simulink model "model_file_sim"  (R2025b)
settings: Solver=ode4  StartTime=0.0  StopTime=5000  FixedStep=1  RelTol=1e-3
values from neighbouring files (symbols this model uses):
  Rc_alu = 10    [modele_valeur.m]
  Rc_fan = 1.2/2    (= 0.6)    [modele_valeur.m]
  Rc_fan1 = 1.2/2    (= 0.6)    [modele_valeur.m]
  Rc_pet = 20/2    (= 10)    [modele_valeur.m]
  Rc_pet1 = 20/2    (= 10)    [modele_valeur.m]
  Rth_alu = 0.1/2    (= 0.05)    [modele_valeur.m]
  Rth_alu2 = 0.1/2    (= 0.05)    [modele_valeur.m]
  Rth_fan = 2.5/2    (= 1.25)    [modele_valeur.m]
  Rth_fan2 = 2.5/2    (= 1.25)    [modele_valeur.m]
  Rth_pet = 5/2    (= 2.5)    [modele_valeur.m]
  Rth_pet2 = 5/2    (= 2.5)    [modele_valeur.m]
  Rth_sen = 24    [modele_valeur.m]
  Rv = 50    [modele_valeur.m]
  Ts = 1    [model_file_elec.m]    (also in modele_valeur.m; thermal_rl_env.m = 0.5)
libraries: fl_lib x34, nesl_utility x6, slpidlib x1, eeAlternativeControllers x1, simulink x1
settings Model: Creator=33683  LastModifiedBy=nael
settings DataIOCC: ExternalInput=data_in  LoadExternalInput=on  SaveOutput=off  SignalLogging=off  DSMLogging=off  SaveTime=off  ReturnWorkspaceOutputs=off
settings SimscapeCC: ExplicitSolverDiagnosticOptions=none

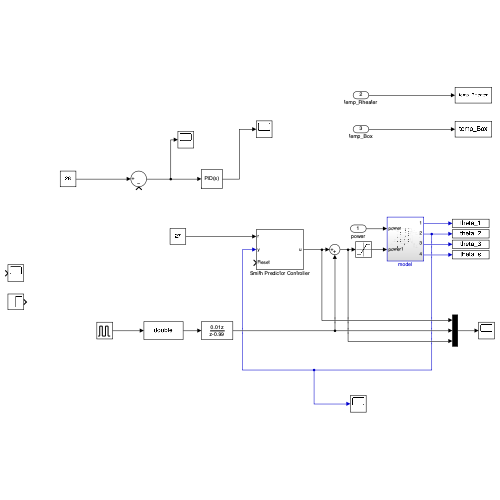
[thumbnail: Simulink's stored preview of the top-level diagram]
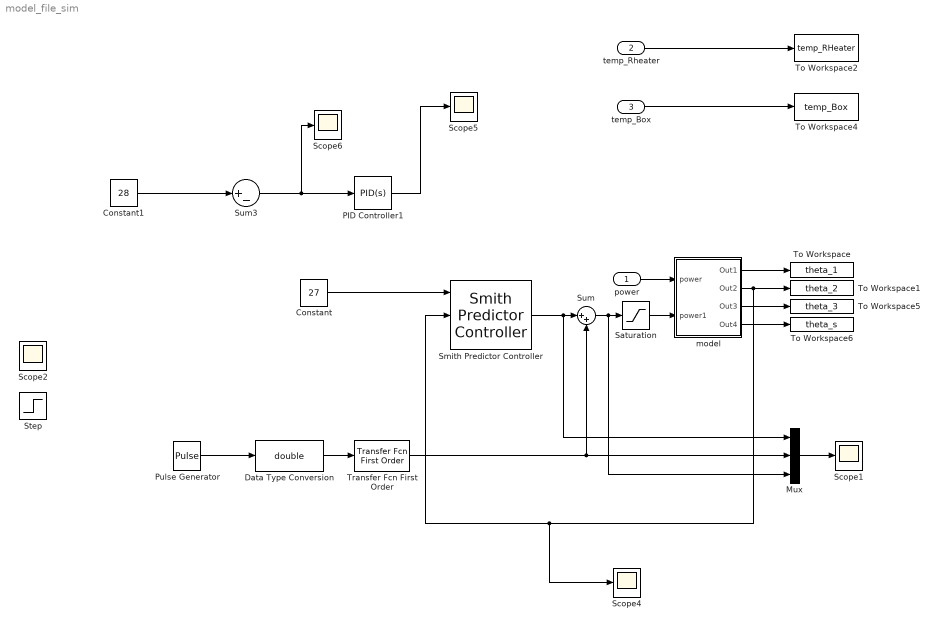
== system model_file_sim ==
  power : Inport
  temp_Rheater : Inport  Port=2
  temp_Box : Inport  Port=3
  Constant : Constant  Value=27
  Constant1 : Constant  Value=28
  Data Type Conversion : DataTypeConversion  OutDataTypeStr=double  SaturateOnIntegerOverflow=off  RndMeth=Floor
  Mux : Mux  Inputs=3
  PID Controller1 : slpidlib/PID Controller  Controller=PID  Form=Parallel  TimeDomain=Continuous-time  UseExternalTs=off  SampleTime=Ts  IntegratorMethod=Forward Euler  FilterMethod=Forward Euler  ControllerParametersSource=internal  P=3  I=0.05  UseKiTs=off  D=0  UseExternalDerivativeSource=off  N=10  UseFilter=on  TunerSelectOption=Transfer Function Based (PID Tuner App)  InitialConditionSource=internal  InitialConditionForIntegrator=0  InitialConditionForFilter=0  DifferentiatorICPrevScaledInput=0  ExternalReset=none  TrackingMode=off  Kt=1  LimitOutput=off  SatLimitsSource=internal  UpperSaturationLimit=inf  LowerSaturationLimit=-inf  LinearizeAsGain=on  AntiWindupMode=none  Kb=1  LimitIntegrator=off  UpperIntegratorSaturationLimit=inf  LowerIntegratorSaturationLimit=-inf  POutMin=[]  POutMax=[]  IOutMin=[]  IOutMax=[]  DOutMin=[]  DOutMax=[]  NOutMin=[]  NOutMax=[]  SumOutMin=[]  SumOutMax=[]  SaturationOutMin=[]  SaturationOutMax=[]  PParamMin=[]  PParamMax=[]  IParamMin=[]  IParamMax=[]  DParamMin=[]  DParamMax=[]  NParamMin=[]  NParamMax=[]  KbParamMin=[]  KbParamMax=[]  KtParamMin=[]  KtParamMax=[]  KbOutMin=[]  KbOutMax=[]  KtOutMin=[]  KtOutMax=[]  IntegratorOutMin=[]  IntegratorOutMax=[]  FilterOutMin=[]  FilterOutMax=[]  SumI1OutMin=[]  SumI1OutMax=[]  SumI2OutMin=[]  SumI2OutMax=[]  SumI3OutMin=[]  SumI3OutMax=[]  SumI4OutMin=[]  SumI4OutMax=[]  SumDOutMin=[]  SumDOutMax=[]  DifferentiatorOutMin=[]  DifferentiatorOutMax=[]  FilterDiffOutCoefMin=[]  FilterDiffOutCoefMax=[]  ReciprocalOutMin=[]  ReciprocalOutMax=[]  SumDenOutMin=[]  SumDenOutMax=[]  SumNumOutMin=[]  SumNumOutMax=[]  DivideOutMin=[]  DivideOutMax=[]  UdiffTsProdOutMin=[]  UdiffTsProdOutMax=[]  NTsProdOutMin=[]  NTsProdOutMax=[]  UintegralTsProdOutMin=[]  UintegralTsProdOutMax=[]  UngainTsProdOutMin=[]  UngainTsProdOutMax=[]  ClampingZeroOutDataTypeStr=Inherit: Inherit via back propagation  ClampingZeroOutMin=[]  ClampingZeroOutMax=[]  FilterDenConstantOutDataTypeStr=Inherit: Inherit via back propagation  FilterDenConstantOutMin=[]  FilterDenConstantOutMax=[]  PCopyOutDataTypeStr=Inherit: Inherit via back propagation  PCopyOutMin=[]  PCopyOutMax=[]  NCopyOutDataTypeStr=Inherit: Inherit via back propagation  NCopyOutMin=[]  NCopyOutMax=[]  IntegratorContinuousStateAttributes=''  IntegratorStateMustResolveToSignalObject=off  IntegratorRTWStateStorageClass=Auto  FilterContinuousStateAttributes=''  FilterStateMustResolveToSignalObject=off  FilterRTWStateStorageClass=Auto  ParallelPVariant=InternalParameters  IdealPVariant=Disabled  IVariant=InternalParameters  DVariant=InternalParameters  IntegratorVariant=Continuous  SatVariant=Disabled  AWVariant=Passthrough  PCopyVariant=Disabled  TRVariant=Disabled  FdbkBlocksVariant=Forward  IdealPFdbkVariant=Disabled  SatFdbkVariant=Disabled  DerivativeFilterVariant=ContFilter  NVariant=InternalParameters  NCopyVariant=Disabled  FilterICVariant=InternalICsFilter  IntegratorICVariant=InternalICs  ExternalResetVariant=Disabled  TRSumVariant=Passthrough  SumFdbkVariant=Disabled  SumVariant=Sum_PID  TsampFilterVariant=InternalTs  TsampNgainVariant=Passthrough  TsampIntegralVariant=Disabled_SignalSpec  ExternalSaturationOutDataTypeStr=Inherit: Same as second input  DerivativeSourceVariant=ErrorSignal  PreIntVariant=InternalPreInt
  Pulse Generator : DiscretePulseGenerator  PulseType=Time based  Amplitude=2  Period=100  PulseWidth=20  PhaseDelay=100
  Saturation : Saturate  UpperLimit=50  LowerLimit=0
  Scope{1..2,4..6} (5 alike) : Scope
      Scope1 settings: ActiveDisplayYMinimum=-0.696783783226232  ActiveDisplayYMaximum=6.2710540490360893  DataLoggingVariableName=ScopeData2
      Scope2 settings: ActiveDisplayYMinimum=-3.19147364275E+6  ActiveDisplayYMaximum=2.865654132791E+7
      Scope4 settings: ActiveDisplayYMinimum=21.349467164172967  ActiveDisplayYMaximum=27.854795522443293
      Scope5 settings: ActiveDisplayYMinimum=-12.29216  ActiveDisplayYMaximum=133.10616  DataLoggingVariableName=ScopeData3
      Scope6 settings: ActiveDisplayYMinimum=-3.6781  ActiveDisplayYMaximum=7.07534  DataLoggingVariableName=ScopeData5
  Smith Predictor Controller : eeAlternativeControllers/Smith Predictor Controller  Kp=3  Ki=0.05  x0=0  B=5  A=0  numd=b  dend=a  d=1  Ts=Ts
      settings: LibrarySourceBlock=ee_sl_lib/General Control/Smith Predictor Controller
  Step : Step  Time=100  After=5  SampleTime=0
  Sum : Sum  Inputs=|++
  Sum3 : Sum  Inputs=|+-
  To Workspace : ToWorkspace  VariableName=theta_1  SampleTime=Ts
  To Workspace1 : ToWorkspace  VariableName=theta_2  SampleTime=Ts
  To Workspace2 : ToWorkspace  VariableName=temp_RHeater  SampleTime=Ts
  To Workspace4 : ToWorkspace  VariableName=temp_Box  SampleTime=Ts
  To Workspace5 : ToWorkspace  VariableName=theta_3  SampleTime=Ts
  To Workspace6 : ToWorkspace  VariableName=theta_s  SampleTime=Ts
  Transfer Fcn First Order : simulink/Discrete/Transfer Fcn First Order  PoleZ=0.99  ICPrevOutput=0.0  DoSatur=off
  model : Subsystem
  wires:
  temp_Rheater/1 -> To Workspace2/1
  temp_Box/1 -> To Workspace4/1
  model/1(Out1) -> To Workspace/1
  model/2(Out2) -> Scope4/1, Smith Predictor Controller/2, To Workspace1/1
  model/3(Out3) -> To Workspace5/1
  model/4(Out4) -> To Workspace6/1
  Sum3/1 -> Scope6/1, PID Controller1/1
  Constant/1 -> Smith Predictor Controller/1
  Constant1/1 -> Sum3/1
  PID Controller1/1 -> Scope5/1
  power/1 -> model/1(power)
  Sum/1 -> Mux/3, Saturation/1
  Mux/1 -> Scope1/1
  Transfer Fcn First Order/1 -> Sum/2, Mux/2
  Pulse Generator/1 -> Data Type Conversion/1
  Data Type Conversion/1 -> Transfer Fcn First Order/1
  Smith Predictor Controller/1 -> Mux/1, Sum/1
  Saturation/1 -> model/2(power1)

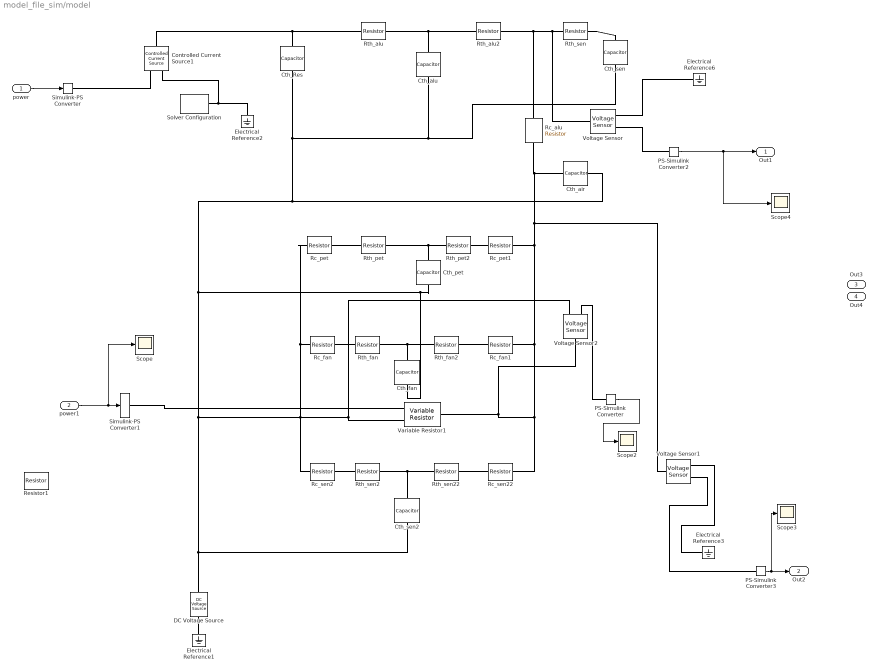
== system model_file_sim/model ==
  power : Inport
  power1 : Inport  Port=2
  Controlled Current Source1 : fl_lib/Electrical/Electrical Sources/Controlled Current Source
  Cth_Res : fl_lib/Electrical/Electrical Elements/Capacitor  c=Cth_Res F  r=0 Ohm  g=0 1/Ohm  i_specify=off  i_priority=None  i=0 A  i_nominal_specify=off  i_nominal_value=1  i_nominal_unit=A  v_specify=off  v_priority=None  v=0 V  v_nominal_specify=off  v_nominal_value=1  v_nominal_unit=V  vc_specify=off  vc_priority=High  vc=0 V  vc_nominal_specify=off  vc_nominal_value=1  vc_nominal_unit=V
  Cth_air : fl_lib/Electrical/Electrical Elements/Capacitor  c=Cth_air F  r=0 Ohm  g=0 1/Ohm  i_specify=off  i_priority=None  i=0 A  i_nominal_specify=off  i_nominal_value=1  i_nominal_unit=A  v_specify=off  v_priority=None  v=0 V  v_nominal_specify=off  v_nominal_value=1  v_nominal_unit=V  vc_specify=off  vc_priority=High  vc=0 V  vc_nominal_specify=off  vc_nominal_value=1  vc_nominal_unit=V
  Cth_alu : fl_lib/Electrical/Electrical Elements/Capacitor  c=Cth_alu F  r=0 Ohm  g=0 1/Ohm  i_specify=off  i_priority=None  i=0 A  i_nominal_specify=off  i_nominal_value=1  i_nominal_unit=A  v_specify=off  v_priority=None  v=0 V  v_nominal_specify=off  v_nominal_value=1  v_nominal_unit=V  vc_specify=off  vc_priority=High  vc=0 V  vc_nominal_specify=off  vc_nominal_value=1  vc_nominal_unit=V
  Cth_fan : fl_lib/Electrical/Electrical Elements/Capacitor  c=Cth_fan F  r=0 Ohm  g=0 1/Ohm  i_specify=off  i_priority=None  i=0 A  i_nominal_specify=off  i_nominal_value=1  i_nominal_unit=A  v_specify=off  v_priority=None  v=0 V  v_nominal_specify=off  v_nominal_value=1  v_nominal_unit=V  vc_specify=off  vc_priority=High  vc=0 V  vc_nominal_specify=off  vc_nominal_value=1  vc_nominal_unit=V
  Cth_pet : fl_lib/Electrical/Electrical Elements/Capacitor  c=Cth_pet F  r=0 Ohm  g=0 1/Ohm  i_specify=off  i_priority=None  i=0 A  i_nominal_specify=off  i_nominal_value=1  i_nominal_unit=A  v_specify=off  v_priority=None  v=0 V  v_nominal_specify=off  v_nominal_value=1  v_nominal_unit=V  vc_specify=off  vc_priority=High  vc=0 V  vc_nominal_specify=off  vc_nominal_value=1  vc_nominal_unit=V
  Cth_sen : fl_lib/Electrical/Electrical Elements/Capacitor  c=Cth_sen F  r=0 Ohm  g=0 1/Ohm  i_specify=off  i_priority=None  i=0 A  i_nominal_specify=off  i_nominal_value=1  i_nominal_unit=A  v_specify=off  v_priority=None  v=0 V  v_nominal_specify=off  v_nominal_value=1  v_nominal_unit=V  vc_specify=off  vc_priority=High  vc=0 V  vc_nominal_specify=off  vc_nominal_value=1  vc_nominal_unit=V
  Cth_sen2 : fl_lib/Electrical/Electrical Elements/Capacitor  c=Cth_pet F  r=0 Ohm  g=0 1/Ohm  i_specify=off  i_priority=None  i=0 A  i_nominal_specify=off  i_nominal_value=1  i_nominal_unit=A  v_specify=off  v_priority=None  v=0 V  v_nominal_specify=off  v_nominal_value=1  v_nominal_unit=V  vc_specify=off  vc_priority=High  vc=0 V  vc_nominal_specify=off  vc_nominal_value=1  vc_nominal_unit=V
  DC Voltage Source : fl_lib/Electrical/Electrical Sources/DC Voltage Source  v0=22 V
  Electrical Reference{1..3,6} (4 alike) : fl_lib/Electrical/Electrical Elements/Electrical Reference
  PS-Simulink Converter : nesl_utility/PS-Simulink Converter  PhysicalDomain=network_engine_domain  SubClassName=ps_output  LeftPortType=input  RightPortType=output  PseudoPeriodic=off  Frequencies=[]  VectorFormat=inherit  Unit=inherit  AffineConversion=off
  PS-Simulink Converter2 : nesl_utility/PS-Simulink Converter  PhysicalDomain=network_engine_domain  SubClassName=ps_output  LeftPortType=input  RightPortType=output  PseudoPeriodic=off  Frequencies=[]  VectorFormat=inherit  Unit=inherit  AffineConversion=off
  PS-Simulink Converter3 : nesl_utility/PS-Simulink Converter  PhysicalDomain=network_engine_domain  SubClassName=ps_output  LeftPortType=input  RightPortType=output  PseudoPeriodic=off  Frequencies=[]  VectorFormat=inherit  Unit=inherit  AffineConversion=off
  Rc_alu : fl_lib/Electrical/Electrical Elements/Resistor  R=Rc_alu Ohm  i_specify=off  i_priority=None  i=0 A  i_nominal_specify=off  i_nominal_value=1  i_nominal_unit=A  v_specify=off  v_priority=None  v=0 V  v_nominal_specify=off  v_nominal_value=1  v_nominal_unit=V
  Rc_fan : fl_lib/Electrical/Electrical Elements/Resistor  R=Rc_fan Ohm  i_specify=off  i_priority=None  i=0 A  i_nominal_specify=off  i_nominal_value=1  i_nominal_unit=A  v_specify=off  v_priority=None  v=0 V  v_nominal_specify=off  v_nominal_value=1  v_nominal_unit=V
  Rc_fan1 : fl_lib/Electrical/Electrical Elements/Resistor  R=Rc_fan1 Ohm  i_specify=off  i_priority=None  i=0 A  i_nominal_specify=off  i_nominal_value=1  i_nominal_unit=A  v_specify=off  v_priority=None  v=0 V  v_nominal_specify=off  v_nominal_value=1  v_nominal_unit=V
  Rc_pet : fl_lib/Electrical/Electrical Elements/Resistor  R=Rc_pet Ohm  i_specify=off  i_priority=None  i=0 A  i_nominal_specify=off  i_nominal_value=1  i_nominal_unit=A  v_specify=off  v_priority=None  v=0 V  v_nominal_specify=off  v_nominal_value=1  v_nominal_unit=V
  Rc_pet1 : fl_lib/Electrical/Electrical Elements/Resistor  R=Rc_pet1 Ohm  i_specify=off  i_priority=None  i=0 A  i_nominal_specify=off  i_nominal_value=1  i_nominal_unit=A  v_specify=off  v_priority=None  v=0 V  v_nominal_specify=off  v_nominal_value=1  v_nominal_unit=V
  Rc_sen2 : fl_lib/Electrical/Electrical Elements/Resistor  R=Rc_fan Ohm  i_specify=off  i_priority=None  i=0 A  i_nominal_specify=off  i_nominal_value=1  i_nominal_unit=A  v_specify=off  v_priority=None  v=0 V  v_nominal_specify=off  v_nominal_value=1  v_nominal_unit=V
  Rc_sen22 : fl_lib/Electrical/Electrical Elements/Resistor  R=Rth_fan Ohm  i_specify=off  i_priority=None  i=0 A  i_nominal_specify=off  i_nominal_value=1  i_nominal_unit=A  v_specify=off  v_priority=None  v=0 V  v_nominal_specify=off  v_nominal_value=1  v_nominal_unit=V
  Resistor1 : fl_lib/Electrical/Electrical Elements/Resistor  R=Rv Ohm  i_specify=off  i_priority=None  i=0 A  i_nominal_specify=off  i_nominal_value=1  i_nominal_unit=A  v_specify=off  v_priority=None  v=0 V  v_nominal_specify=off  v_nominal_value=1  v_nominal_unit=V
  Rth_alu : fl_lib/Electrical/Electrical Elements/Resistor  R=Rth_alu Ohm  i_specify=off  i_priority=None  i=0 A  i_nominal_specify=off  i_nominal_value=1  i_nominal_unit=A  v_specify=off  v_priority=None  v=0 V  v_nominal_specify=off  v_nominal_value=1  v_nominal_unit=V
  Rth_alu2 : fl_lib/Electrical/Electrical Elements/Resistor  R=Rth_alu2 Ohm  i_specify=off  i_priority=None  i=0 A  i_nominal_specify=off  i_nominal_value=1  i_nominal_unit=A  v_specify=off  v_priority=None  v=0 V  v_nominal_specify=off  v_nominal_value=1  v_nominal_unit=V
  Rth_fan : fl_lib/Electrical/Electrical Elements/Resistor  R=Rth_fan Ohm  i_specify=off  i_priority=None  i=0 A  i_nominal_specify=off  i_nominal_value=1  i_nominal_unit=A  v_specify=off  v_priority=None  v=0 V  v_nominal_specify=off  v_nominal_value=1  v_nominal_unit=V
  Rth_fan2 : fl_lib/Electrical/Electrical Elements/Resistor  R=Rth_fan2 Ohm  i_specify=off  i_priority=None  i=0 A  i_nominal_specify=off  i_nominal_value=1  i_nominal_unit=A  v_specify=off  v_priority=None  v=0 V  v_nominal_specify=off  v_nominal_value=1  v_nominal_unit=V
  Rth_pet : fl_lib/Electrical/Electrical Elements/Resistor  R=Rth_pet Ohm  i_specify=off  i_priority=None  i=0 A  i_nominal_specify=off  i_nominal_value=1  i_nominal_unit=A  v_specify=off  v_priority=None  v=0 V  v_nominal_specify=off  v_nominal_value=1  v_nominal_unit=V
  Rth_pet2 : fl_lib/Electrical/Electrical Elements/Resistor  R=Rth_pet2 Ohm  i_specify=off  i_priority=None  i=0 A  i_nominal_specify=off  i_nominal_value=1  i_nominal_unit=A  v_specify=off  v_priority=None  v=0 V  v_nominal_specify=off  v_nominal_value=1  v_nominal_unit=V
  Rth_sen : fl_lib/Electrical/Electrical Elements/Resistor  R=Rth_sen Ohm  i_specify=off  i_priority=None  i=0 A  i_nominal_specify=off  i_nominal_value=1  i_nominal_unit=A  v_specify=off  v_priority=None  v=0 V  v_nominal_specify=off  v_nominal_value=1  v_nominal_unit=V
  Rth_sen2 : fl_lib/Electrical/Electrical Elements/Resistor  R=Rth_fan Ohm  i_specify=off  i_priority=None  i=0 A  i_nominal_specify=off  i_nominal_value=1  i_nominal_unit=A  v_specify=off  v_priority=None  v=0 V  v_nominal_specify=off  v_nominal_value=1  v_nominal_unit=V
  Rth_sen22 : fl_lib/Electrical/Electrical Elements/Resistor  R=Rc_fan Ohm  i_specify=off  i_priority=None  i=0 A  i_nominal_specify=off  i_nominal_value=1  i_nominal_unit=A  v_specify=off  v_priority=None  v=0 V  v_nominal_specify=off  v_nominal_value=1  v_nominal_unit=V
  Scope{,2..4} (4 alike) : Scope
      Scope settings: ActiveDisplayYMinimum=1.1179174747738359  ActiveDisplayYMaximum=6.0694205759249709
      Scope2 settings: ActiveDisplayYMinimum=-0.6454786667977801  ActiveDisplayYMaximum=5.809308001180022
      Scope3 settings: ActiveDisplayYMinimum=21.048786988457906  ActiveDisplayYMaximum=30.56091710387885  DataLoggingVariableName=ScopeData2
      Scope4 settings: ActiveDisplayYMinimum=14.19123  ActiveDisplayYMaximum=92.27893  DataLoggingVariableName=ScopeData4
  Simulink-PS Converter : nesl_utility/Simulink-PS Converter  PhysicalDomain=network_engine_domain  SubClassName=ps_input  LeftPortType=input  RightPortType=output  PseudoPeriodic=off  Frequencies=[]  NoiseDistribution=none  NoiseParameters=[]  Unit=1  AffineConversion=off  FilteringAndDerivatives=provide  SimscapeFilterOrder=1  InputFilterTimeConstant=0.001  UdotUserProvided=0
  Simulink-PS Converter1 : nesl_utility/Simulink-PS Converter  PhysicalDomain=network_engine_domain  SubClassName=ps_input  LeftPortType=input  RightPortType=output  PseudoPeriodic=off  Frequencies=[]  NoiseDistribution=none  NoiseParameters=[]  Unit=V/A  AffineConversion=off  FilteringAndDerivatives=filter  SimscapeFilterOrder=1  InputFilterTimeConstant=Ts  UdotUserProvided=0
  Solver Configuration : nesl_utility/Solver Configuration  PhysicalDomain=network_engine_domain  SubClassName=solver  LeftPortType=input  RightPortType=generic  Tones=[]  Harmonics=[]  SimulateNoise=off  Profile=off  UseLocalSampling=off  EnableSwitchedLinearOptims=on  FrequencyDomain=off  UseCCode=off  RelTol=0.001  AbsTol=0.001  MinStep=1e-09  ToWorkspace=off  RevertToSquareIcSolve=off  NumHomotopyIterations=100  PhasorMode=off  PhasorModeNumHarmonics=1  ConsistencySolver=NEWTON_XTOL_AFTER_FTOL  IndexReductionMethod=DerivativeReplacement  DoDC=off  ResidualTolerance=1e-09  ConsistencyTolSource=GLOBAL  ConsistencyAbsTol=0.001  ConsistencyRelTol=0.001  ConsistencyTolFactor=0.001  UseLocalSolver=off  LocalSolverChoice=NE_BACKWARD_EULER_ADVANCER  ResolveIndetEquations=on  FunctionEvalNumThread=1  LocalSolverSampleTime=0.001  DoFixedCost=off  MaxNonlinIter=3  MaxModeIter=2  ComputeImpulses=off  ImpulseIterations=2  LinearAlgebra=auto  LinearAlgebraNumThread=0  EquationFormulation=NE_TIME_EF  DelaysMemoryBudget=1024  AutomaticFiltering=on  FilteringTimeConstant=0.001  PartitionStorageMethod=AS_NEEDED  PartitionMemoryBudget=1024  PartitionMethod=ROBUST  MultibodyUseLocalSolver=off  MultibodyLocalSolverChoice=ODE1  MultibodyLocalSolverSampleTime=0.001
  Variable Resistor1 : fl_lib/Electrical/Electrical Elements/Variable Resistor  Rmin=0.2 Ohm  thermalEnable=false  thermal_mass=1 J/K  i_specify=off  i_priority=None  i=0 A  i_nominal_specify=off  i_nominal_value=1  i_nominal_unit=A  v_specify=off  v_priority=None  v=0 V  v_nominal_specify=off  v_nominal_value=1  v_nominal_unit=V  T_specify=off  T_priority=None  T=300 K  T_nominal_specify=off  T_nominal_value=1  T_nominal_unit=K
  Voltage Sensor : fl_lib/Electrical/Electrical Sensors/Voltage Sensor
  Voltage Sensor1 : fl_lib/Electrical/Electrical Sensors/Voltage Sensor
  Voltage Sensor2 : fl_lib/Electrical/Electrical Sensors/Voltage Sensor
  Out1 : Outport
  Out2 : Outport  Port=2
  Out3 : Outport  Port=3
  Out4 : Outport  Port=4
  wires:
  PS-Simulink Converter3/1 -> Scope3/1, Out2/1
  PS-Simulink Converter2/1 -> Scope4/1, Out1/1
  power/1 -> Simulink-PS Converter/1
  PS-Simulink Converter/1 -> Scope2/1
  power1/1 -> Scope/1, Simulink-PS Converter1/1
  connections:
  Cth_Res/RConn1 -- Cth_sen/RConn1 -- Cth_alu/RConn1 -- Cth_air/RConn1 -- Cth_fan/RConn1 -- Cth_pet/RConn1 -- DC Voltage Source/LConn1 -- Cth_sen2/RConn1 -- Variable Resistor1/LConn2 -- Voltage Sensor2/RConn2 -- Rc_sen2/LConn1 -- Rc_pet/LConn1 -- Rc_fan/LConn1
  Voltage Sensor/LConn1 -- Rth_alu2/RConn1 -- Rc_alu/LConn1 -- Rth_sen/LConn1
  Rth_pet/RConn1 -- Cth_pet/LConn1 -- Rth_pet2/LConn1
  Rth_fan2/LConn1 -- Cth_fan/LConn1 -- Rth_fan/RConn1
  Cth_alu/LConn1 -- Rth_alu2/LConn1 -- Rth_alu/RConn1
  Cth_Res/LConn1 -- Controlled Current Source1/LConn1 -- Rth_alu/LConn1
  Solver Configuration/RConn1 -- Controlled Current Source1/RConn2 -- Electrical Reference2/LConn1
  Rth_sen22/LConn1 -- Rth_sen2/RConn1 -- Cth_sen2/LConn1
  Electrical Reference3/LConn1 -- Voltage Sensor1/RConn2
  DC Voltage Source/RConn1 -- Electrical Reference1/LConn1
  Rth_sen/RConn1 -- Cth_sen/LConn1
  Rth_pet/LConn1 -- Rc_pet/RConn1
  Voltage Sensor1/RConn1 -- PS-Simulink Converter3/LConn1
  Rth_fan/LConn1 -- Rc_fan/RConn1
  Rth_sen2/LConn1 -- Rc_sen2/RConn1
  Controlled Current Source1/RConn1 -- Simulink-PS Converter/RConn1
  Electrical Reference6/LConn1 -- Voltage Sensor/RConn2
  Rc_sen22/LConn1 -- Rth_sen22/RConn1
  Rc_fan1/LConn1 -- Rth_fan2/RConn1
  Voltage Sensor/RConn1 -- PS-Simulink Converter2/LConn1
  Rc_pet1/LConn1 -- Rth_pet2/RConn1
  Voltage Sensor1/LConn1 -- Cth_air/LConn1 -- Rc_alu/RConn1 -- Rc_pet1/RConn1 -- Rc_fan1/RConn1 -- Rc_sen22/RConn1 -- Variable Resistor1/RConn1 -- Voltage Sensor2/LConn1
  Voltage Sensor2/RConn1 -- PS-Simulink Converter/LConn1
  Variable Resistor1/LConn1 -- Simulink-PS Converter1/RConn1
